simulink model "cubesat_adcs_pid_yay"  (R2026b)
settings: Solver=VariableStepAuto  StopTime=150.0
settings Model: Creator=Adyanshu  LastModifiedBy=Adyanshu

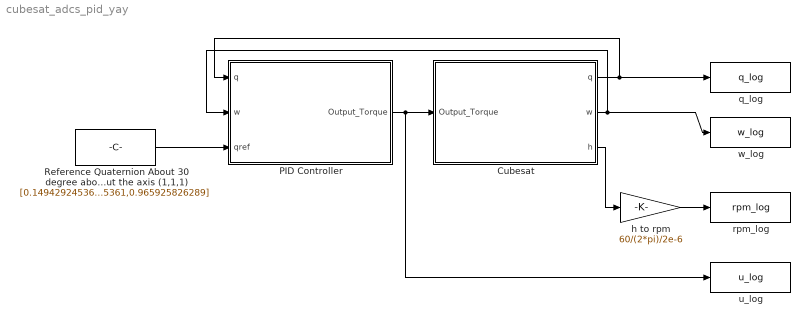
== system cubesat_adcs_pid_yay ==
  Cubesat : Subsystem
  PID Controller : Subsystem
  Reference Quaternion About 30 degree about the axis (1,1,1) : Constant  Value=[0.149429245361,0.149429245361,0.149429245361,0.965925826289]
  h to rpm : Gain  Gain=60/(2*pi)/2e-6
  q_log : ToWorkspace  VariableName=q_log  SaveFormat=Timeseries  SampleTime=-1
  rpm_log : ToWorkspace  VariableName=rpm_log  SaveFormat=Timeseries  SampleTime=-1
  u_log : ToWorkspace  VariableName=u_log  SaveFormat=Timeseries  SampleTime=-1
  w_log : ToWorkspace  VariableName=w_log  SaveFormat=Timeseries  SampleTime=-1
  wires:
  Reference Quaternion About 30 degree about the axis (1,1,1)/1 -> PID Controller/3(qref)
  Cubesat/1(q) -> q_log/1, PID Controller/1(q)
  Cubesat/2(w) -> PID Controller/2(w), w_log/1
  h to rpm/1 -> rpm_log/1
  Cubesat/3(h) -> h to rpm/1
  PID Controller/1(Output_Torque) -> u_log/1, Cubesat/1(Output_Torque)

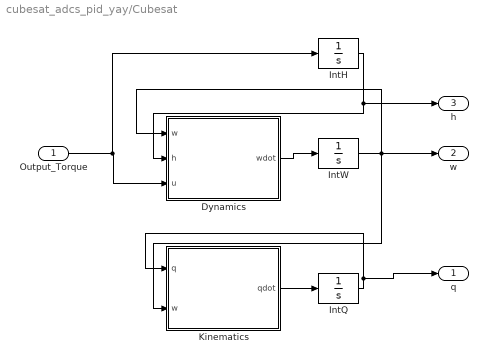
== system cubesat_adcs_pid_yay/Cubesat ==
  Output_Torque : Inport
  Dynamics : MATLAB Function  TreatAsAtomicUnit=on
  IntH : Integrator  InitialCondition=zeros(3,1)
  IntQ : Integrator  InitialCondition=[1; 0; 0; 0]
  IntW : Integrator  InitialCondition=[0.02; -0.01; 0.015]
  Kinematics : MATLAB Function  TreatAsAtomicUnit=on
  q : Outport
  w : Outport  Port=2
  h : Outport  Port=3
  wires:
  Output_Torque/1 -> Dynamics/3(u), IntH/1
  IntH/1 -> Dynamics/2(h), h/1
  Dynamics/1(wdot) -> IntW/1
  IntW/1 -> Kinematics/2(w), Dynamics/1(w), w/1
  Kinematics/1(qdot) -> IntQ/1
  IntQ/1 -> Kinematics/1(q), q/1

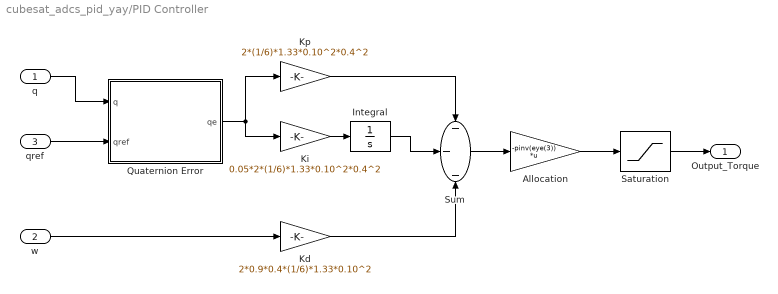
== system cubesat_adcs_pid_yay/PID Controller ==
  q : Inport
  w : Inport  Port=2
  qref : Inport  Port=3
  Allocation : Gain  Gain=-pinv(eye(3))  Multiplication=Matrix(K*u)
  Integral : Integrator  InitialCondition=zeros(3,1)  LimitOutput=on  UpperSaturationLimit=0.1  LowerSaturationLimit=-0.1
  Kd : Gain  Gain=2*0.9*0.4*(1/6)*1.33*0.10^2
  Ki : Gain  Gain=0.05*2*(1/6)*1.33*0.10^2*0.4^2
  Kp : Gain  Gain=2*(1/6)*1.33*0.10^2*0.4^2
  Quaternion Error : MATLAB Function  TreatAsAtomicUnit=on
  Saturation : Saturate  UpperLimit=2e-3  LowerLimit=-2e-3
  Sum : Sum  Inputs=---
  Output_Torque : Outport
  wires:
  q/1 -> Quaternion Error/1(q)
  qref/1 -> Quaternion Error/2(qref)
  Quaternion Error/1(qe) -> Kp/1, Ki/1
  Ki/1 -> Integral/1
  w/1 -> Kd/1
  Kp/1 -> Sum/1
  Integral/1 -> Sum/2
  Kd/1 -> Sum/3
  Sum/1 -> Allocation/1
  Allocation/1 -> Saturation/1
  Saturation/1 -> Output_Torque/1

== matlab function cubesat_adcs_pid_yay/Cubesat/Dynamics ==
  data: w input; h input; u input; wdot output
function wdot = Dynamics(w, h, u)
% I*wdot = -u - cross(w, I*w + h)
I = diag([0.002216666667 0.002216666667 0.002216666667]);
wdot = I \ ( -u - cross(w, I*w + h) );
end

== matlab function cubesat_adcs_pid_yay/Cubesat/Kinematics ==
  data: q input; qdot output; w input
function qdot = Kinematics(q, w)
M = [-q(2) -q(3) -q(4);
      q(1) -q(4)  q(3);
      q(4)  q(1) -q(2);
     -q(3)  q(2)  q(1)];
k = 1;  % keeps magnitude of q = 1 against numerical drift
qdot = 0.5*M*w + k*(1 - (q'*q))*q;
end

== matlab function cubesat_adcs_pid_yay/PID Controller/Quaternion Error ==
  data: q input; qe output; qref input
function qe = QuatError(q, qref)
% Error quaternion qe = conj(qd) * q (scalar-first)
e0 = qref(1)*q(1) + qref(2)*q(2) + qref(3)*q(3) + qref(4)*q(4);
e1 = qref(1)*q(2) - qref(2)*q(1) - qref(3)*q(4) + qref(4)*q(3);
e2 = qref(1)*q(3) + qref(2)*q(4) - qref(3)*q(1) - qref(4)*q(2);
e3 = qref(1)*q(4) - qref(2)*q(3) + qref(3)*q(2) - qref(4)*q(1);
% q and -q are the same rotation: pick the short way around
if e0 < 0, s = -1; else, s = 1; end
qe = s*[e1; e2; e3];
end
